simulink model "test_CHCmdApi1"  (R2023a)
settings: Solver=ode4  StartTime=0.0  StopTime=10.0  FixedStep=0.002  RelTol=1e-3
libraries: AFC5Toolbox x6
settings Model: Creator=zhangr365  LastModifiedBy=zqinghua
settings OptimizationCC: DefaultParameterBehavior=Inlined  EnhancedBackFolding=on  PassReuseOutputArgsAs=Individual arguments  ZeroExternalMemoryAtStartup=off  ZeroInternalMemoryAtStartup=off  OptimizeBlockOrder=speed  DifferentSizesBufferReuse=on  OptimizationCustomize=off  EfficientTunableParamExpr=on
settings DebuggingCC: ParameterTunabilityLossMsg=error
settings HardwareCC: ProdBitPerInt=16  ProdBitPerPointer=16  ProdBitPerSizeT=16  ProdBitPerPtrDiffT=16  ProdLargestAtomicFloat=None  ProdWordSize=16  ProdHWDeviceType=STMicroelectronics->ST10/Super10
settings SFSimCC: MATLABDynamicMemAlloc=off
settings RTWCC: Description=Embedded Coder  SystemTargetFile=AFCHawk.tlc  GenCodeOnly=on  TemplateMakefile=ert_default_tmf
settings CodeAppCC: ForceParamTrailComments=on  IgnoreCustomStorageClasses=off  OperatorAnnotations=on  SimulinkDataObjDesc=on  SFDataObjDesc=on  InsertBlockDesc=on
settings STFCustomTargetCC: MultiwordLength=256  ModelReferenceCompliant=off  ConcurrentExecutionCompliant=off  CombineOutputUpdateFcns=on  ERTCustomFileBanners=on  SupportContinuousTime=off  SupportNonInlinedSFcns=off  RemoveResetFunc=on  MATLABClassNameForMDSCustomization=Simulink.SoftwareTarget.ERTCustomization  GRTInterface=off  UseToolchainInfoCompliant=off  SystemTargetFile=AFCHawk.tlc
settings ERTTargetCC: TargetLangStandard=C99 (ISO)  ModelReferenceCompliant=off  ParMdlRefBuildCompliant=off  CompOptLevelCompliant=off  ConcurrentExecutionCompliant=off  ModelStepFunctionPrototypeControlCompliant=off  CPPClassGenCompliant=off  UseToolchainInfoCompliant=off  InlinedParameterPlacement=NonHierarchical  ERTCustomFileTemplate=example_file_process.tlc

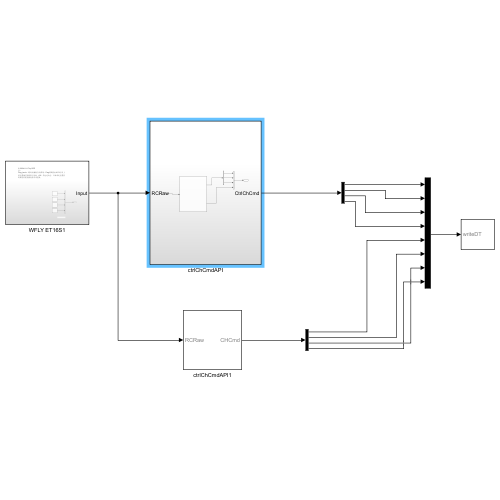
[thumbnail: Simulink's stored preview of the top-level diagram]
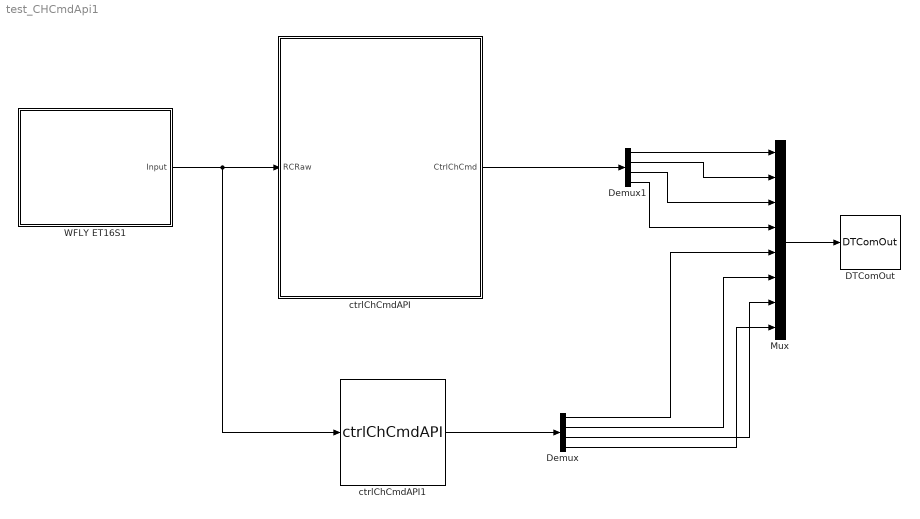
== system test_CHCmdApi1 ==
  DTComOut : AFC5Toolbox/DeviceModule/DTComOut  Priority=8  g_frameType=1  g_outFreq=1  g_comPort=0  g_instName=0  g_id=0
      settings: SourceProductName=AFC5Toolbox
  Demux : Demux
  Demux1 : Demux
  Mux : Mux  Inputs=8
  WFLY ET16S1 : Subsystem  Priority=0
  ctrlChCmdAPI : Subsystem
  ctrlChCmdAPI1 : AFC5Toolbox/APPModule/ctrlChCmdAPI  Priority=3
      settings: SourceProductName=AFC5Toolbox
  wires:
  WFLY ET16S1/1(Input) -> ctrlChCmdAPI1/1, ctrlChCmdAPI/1(RCRaw)
  ctrlChCmdAPI1/1 -> Demux/1
  ctrlChCmdAPI/1(CtrlChCmd) -> Demux1/1
  Demux1/1 -> Mux/1
  Demux1/2 -> Mux/2
  Demux1/3 -> Mux/3
  Demux1/4 -> Mux/4
  Demux/1 -> Mux/5
  Demux/2 -> Mux/6
  Demux/3 -> Mux/7
  Demux/4 -> Mux/8
  Mux/1 -> DTComOut/1

== system test_CHCmdApi1/WFLY ET16S1 ==
  note: cmd4 = [352,1695]
  note: % 2024-01-17 by REZ
      | 注：
      | Flag_land = 1的时候触发自动降落，Flag的跳变由X和Y方向上的位置偏差距离原点坐标（0,0）的远近决定，具体参见位置控制器里的航迹规划指令设置处
  Mux2 : Mux
  SBusCmd{,1..3} (4 alike) : AFC5Toolbox/DeviceModule/SBusCmd  Priority=0  g_SBusChanel=1  g_sampleTime=0.002
      settings: SourceProductName=AFC5Toolbox
  Input : Outport
  wires:
  Mux2/1 -> Input/1
  SBusCmd3/1 -> Mux2/4
  SBusCmd/1 -> Mux2/1
  SBusCmd1/1 -> Mux2/2
  SBusCmd2/1 -> Mux2/3

== system test_CHCmdApi1/ctrlChCmdAPI ==
  RCRaw : Inport
  Demux : Demux  Outputs=3
  Mux : Mux
  get_rccmd_simulink_value : Subsystem
  CtrlChCmd : Outport
  wires:
  RCRaw/1 -> get_rccmd_simulink_value/1(RCRaw)
  get_rccmd_simulink_value/1(RCServCmd) -> Demux/1
  Demux/1 -> Mux/1
  Demux/2 -> Mux/2
  Demux/3 -> Mux/3
  get_rccmd_simulink_value/2(climb_rate) -> Mux/4
  Mux/1 -> CtrlChCmd/1

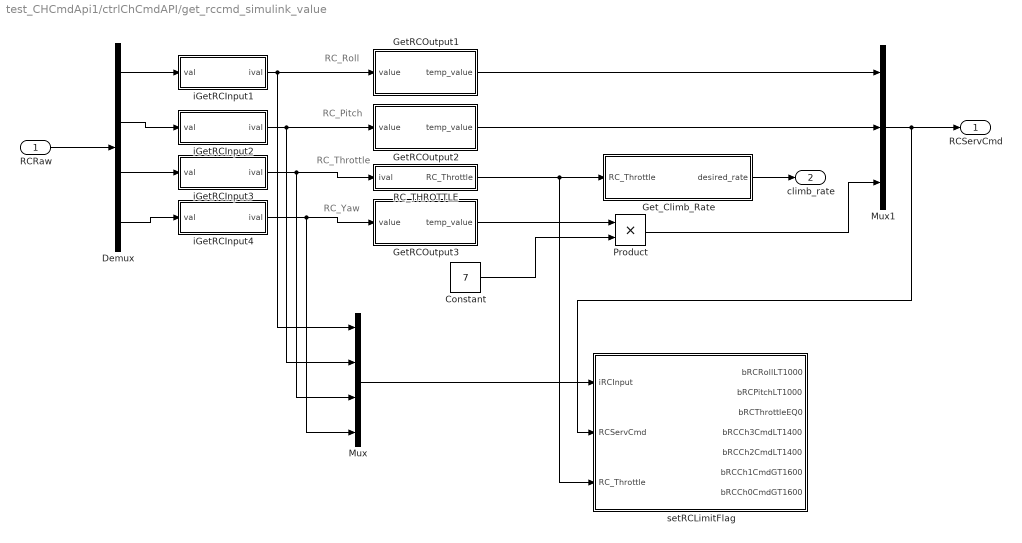
== system test_CHCmdApi1/ctrlChCmdAPI/get_rccmd_simulink_value ==
  note: RC_Roll
  note: RC_Pitch
  note: RC_Yaw
  note: RC_Throttle
  RCRaw : Inport
  Constant : Constant  Value=7
  Demux : Demux
  GetRCOutput1 : Subsystem
  GetRCOutput2 : Subsystem
  GetRCOutput3 : Subsystem
  Get_Climb_Rate : Subsystem
  Mux : Mux
  Mux1 : Mux  Inputs=3
  Product : Product
  RC_THROTTLE : Subsystem
  iGetRCInput1 : Subsystem
  iGetRCInput2 : Subsystem
  iGetRCInput3 : Subsystem
  iGetRCInput4 : Subsystem
  setRCLimitFlag : Subsystem
  RCServCmd : Outport
  climb_rate : Outport  Port=2
  wires:
  Demux/3 -> iGetRCInput3/1(val)
  Demux/4 -> iGetRCInput4/1(val)
  RCRaw/1 -> Demux/1
  Demux/1 -> iGetRCInput1/1(val)
  Mux/1 -> setRCLimitFlag/1(iRCInput)
  GetRCOutput3/1(temp_value) -> Product/1
  Demux/2 -> iGetRCInput2/1(val)
  iGetRCInput4/1(ival) -> Mux/4, GetRCOutput3/1(value)
  iGetRCInput2/1(ival) -> Mux/2, GetRCOutput2/1(value)
  RC_THROTTLE/1(RC_Throttle) -> Get_Climb_Rate/1(RC_Throttle), setRCLimitFlag/3(RC_Throttle)
  iGetRCInput3/1(ival) -> Mux/3, RC_THROTTLE/1(ival)
  Get_Climb_Rate/1(desired_rate) -> climb_rate/1
  iGetRCInput1/1(ival) -> GetRCOutput1/1(value), Mux/1
  Constant/1 -> Product/2
  Product/1 -> Mux1/3
  GetRCOutput1/1(temp_value) -> Mux1/1
  GetRCOutput2/1(temp_value) -> Mux1/2
  Mux1/1 -> RCServCmd/1, setRCLimitFlag/2(RCServCmd)

== system test_CHCmdApi1/ctrlChCmdAPI/get_rccmd_simulink_value/GetRCOutput1 ==
  value : Inport
  If : If  IfExpression=u1 > 1600  ElseIfExpressions=u1 <1400
  If Action Subsystem : Subsystem  TreatAsAtomicUnit=on
  If Action Subsystem1 : Subsystem  TreatAsAtomicUnit=on
  If Action Subsystem2 : Subsystem  TreatAsAtomicUnit=on
  Merge : Merge  Inputs=3
  temp_value : Outport
  wires:
  value/1 -> If Action Subsystem1/1(value), If Action Subsystem/1(value), If/1
  If/1 -> If Action Subsystem/Action
  If/2 -> If Action Subsystem1/Action
  If/3 -> If Action Subsystem2/Action
  If Action Subsystem1/1(temp_value) -> Merge/2
  If Action Subsystem/1(temp_value) -> Merge/1
  If Action Subsystem2/1(temp_value) -> Merge/3
  Merge/1 -> temp_value/1

== system test_CHCmdApi1/ctrlChCmdAPI/get_rccmd_simulink_value/GetRCOutput2 ==
  value : Inport
  If : If  IfExpression=u1 > 1600  ElseIfExpressions=u1 <1400
  If Action Subsystem : Subsystem  TreatAsAtomicUnit=on
  If Action Subsystem1 : Subsystem  TreatAsAtomicUnit=on
  If Action Subsystem2 : Subsystem  TreatAsAtomicUnit=on
  Merge : Merge  Inputs=3
  temp_value : Outport
  wires:
  value/1 -> If Action Subsystem1/1(value), If Action Subsystem/1(value), If/1
  If/1 -> If Action Subsystem/Action
  If/2 -> If Action Subsystem1/Action
  If/3 -> If Action Subsystem2/Action
  If Action Subsystem1/1(temp_value) -> Merge/2
  If Action Subsystem/1(temp_value) -> Merge/1
  If Action Subsystem2/1(temp_value) -> Merge/3
  Merge/1 -> temp_value/1

== system test_CHCmdApi1/ctrlChCmdAPI/get_rccmd_simulink_value/GetRCOutput3 ==
  value : Inport
  If : If  IfExpression=u1 > 1600  ElseIfExpressions=u1 <1400
  If Action Subsystem : Subsystem  TreatAsAtomicUnit=on
  If Action Subsystem1 : Subsystem  TreatAsAtomicUnit=on
  If Action Subsystem2 : Subsystem  TreatAsAtomicUnit=on
  Merge : Merge  Inputs=3
  temp_value : Outport
  wires:
  value/1 -> If Action Subsystem1/1(value), If Action Subsystem/1(value), If/1
  If/1 -> If Action Subsystem/Action
  If/2 -> If Action Subsystem1/Action
  If/3 -> If Action Subsystem2/Action
  If Action Subsystem1/1(temp_value) -> Merge/2
  If Action Subsystem/1(temp_value) -> Merge/1
  If Action Subsystem2/1(temp_value) -> Merge/3
  Merge/1 -> temp_value/1

== system test_CHCmdApi1/ctrlChCmdAPI/get_rccmd_simulink_value/Get_Climb_Rate ==
  RC_Throttle : Inport
  If : If  IfExpression=u1 < 400  ElseIfExpressions=u1 > 600
  If Action Subsystem1 : Subsystem  TreatAsAtomicUnit=on
  If Action Subsystem2 : Subsystem  TreatAsAtomicUnit=on
  If Action Subsystem3 : Subsystem  TreatAsAtomicUnit=on
  Merge : Merge  Inputs=3
  desired_rate : Outport
  wires:
  If Action Subsystem2/1(desired_rate) -> Merge/1
  Merge/1 -> desired_rate/1
  If Action Subsystem3/1(desired_rate) -> Merge/3
  RC_Throttle/1 -> If Action Subsystem2/1(value), If Action Subsystem1/1(value), If/1
  If/1 -> If Action Subsystem2/Action
  If/2 -> If Action Subsystem1/Action
  If/3 -> If Action Subsystem3/Action
  If Action Subsystem1/1(desired_rate) -> Merge/2

== system test_CHCmdApi1/ctrlChCmdAPI/get_rccmd_simulink_value/RC_THROTTLE ==
  ival : Inport
  If : If  IfExpression=u1 < 1100  ElseIfExpressions=u1 > 1900
  If Action Subsystem1 : Subsystem  TreatAsAtomicUnit=on
  If Action Subsystem2 : Subsystem  TreatAsAtomicUnit=on
  If Action Subsystem3 : Subsystem  TreatAsAtomicUnit=on
  Merge : Merge  Inputs=3
  RC_Throttle : Outport
  wires:
  ival/1 -> If Action Subsystem3/1(ival), If/1
  If/1 -> If Action Subsystem2/Action
  If Action Subsystem2/1(RC_Throttle) -> Merge/1
  If/2 -> If Action Subsystem1/Action
  If Action Subsystem1/1(RC_Throttle) -> Merge/2
  If/3 -> If Action Subsystem3/Action
  If Action Subsystem3/1(RC_Throttle) -> Merge/3
  Merge/1 -> RC_Throttle/1

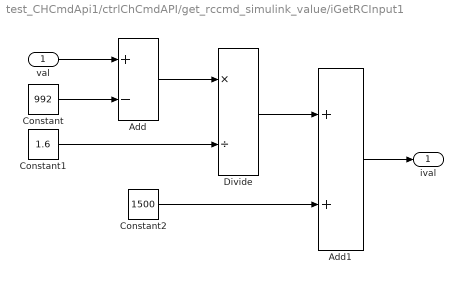
== system test_CHCmdApi1/ctrlChCmdAPI/get_rccmd_simulink_value/iGetRCInput1 ==
  val : Inport
  Add : Sum  Inputs=+-
  Add1 : Sum
  Constant : Constant  Value=992
  Constant1 : Constant  Value=1.6
  Constant2 : Constant  Value=1500
  Divide : Product  Inputs=*/
  ival : Outport
  wires:
  val/1 -> Add/1
  Constant/1 -> Add/2
  Add/1 -> Divide/1
  Constant1/1 -> Divide/2
  Divide/1 -> Add1/1
  Constant2/1 -> Add1/2
  Add1/1 -> ival/1

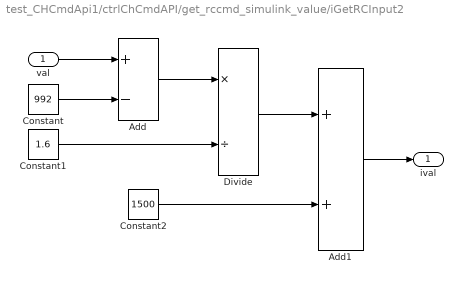
== system test_CHCmdApi1/ctrlChCmdAPI/get_rccmd_simulink_value/iGetRCInput2 ==
  val : Inport
  Add : Sum  Inputs=+-
  Add1 : Sum
  Constant : Constant  Value=992
  Constant1 : Constant  Value=1.6
  Constant2 : Constant  Value=1500
  Divide : Product  Inputs=*/
  ival : Outport
  wires:
  val/1 -> Add/1
  Constant/1 -> Add/2
  Add/1 -> Divide/1
  Constant1/1 -> Divide/2
  Divide/1 -> Add1/1
  Constant2/1 -> Add1/2
  Add1/1 -> ival/1

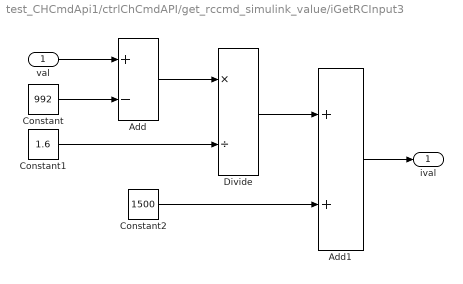
== system test_CHCmdApi1/ctrlChCmdAPI/get_rccmd_simulink_value/iGetRCInput3 ==
  val : Inport
  Add : Sum  Inputs=+-
  Add1 : Sum
  Constant : Constant  Value=992
  Constant1 : Constant  Value=1.6
  Constant2 : Constant  Value=1500
  Divide : Product  Inputs=*/
  ival : Outport
  wires:
  val/1 -> Add/1
  Constant/1 -> Add/2
  Add/1 -> Divide/1
  Constant1/1 -> Divide/2
  Divide/1 -> Add1/1
  Constant2/1 -> Add1/2
  Add1/1 -> ival/1

== system test_CHCmdApi1/ctrlChCmdAPI/get_rccmd_simulink_value/iGetRCInput4 ==
  val : Inport
  Add : Sum  Inputs=+-
  Add1 : Sum
  Constant : Constant  Value=992
  Constant1 : Constant  Value=1.6
  Constant2 : Constant  Value=1500
  Divide : Product  Inputs=*/
  ival : Outport
  wires:
  val/1 -> Add/1
  Constant/1 -> Add/2
  Add/1 -> Divide/1
  Constant1/1 -> Divide/2
  Divide/1 -> Add1/1
  Constant2/1 -> Add1/2
  Add1/1 -> ival/1

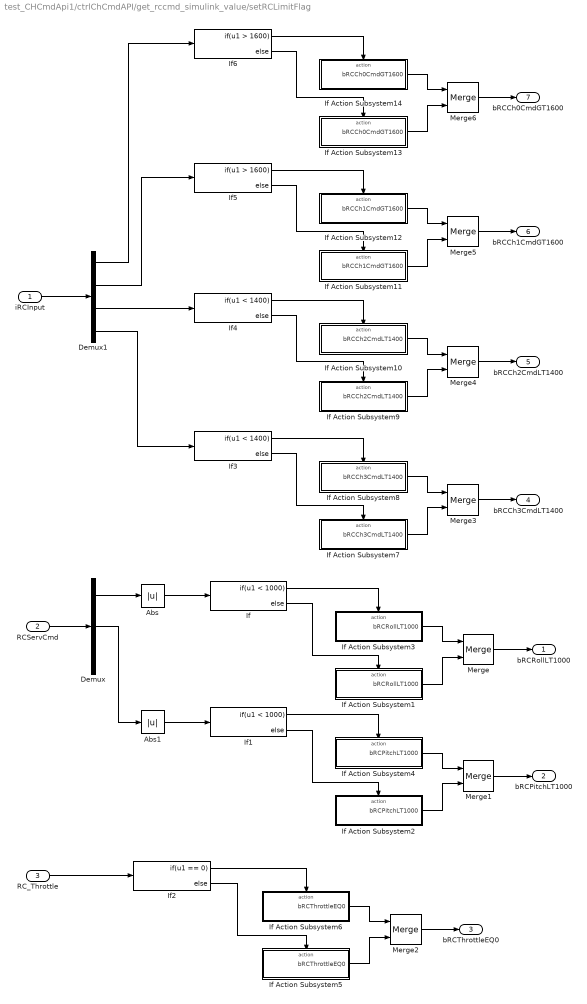
== system test_CHCmdApi1/ctrlChCmdAPI/get_rccmd_simulink_value/setRCLimitFlag ==
  iRCInput : Inport
  RCServCmd : Inport  Port=2
  RC_Throttle : Inport  Port=3
  Abs : Abs  SaturateOnIntegerOverflow=off
  Abs1 : Abs  SaturateOnIntegerOverflow=off
  Demux : Demux  Outputs=3
  Demux1 : Demux
  If : If  IfExpression=u1 < 1000
  If Action Subsystem1 : Subsystem  TreatAsAtomicUnit=on
  If Action Subsystem10 : Subsystem  TreatAsAtomicUnit=on
  If Action Subsystem11 : Subsystem  TreatAsAtomicUnit=on
  If Action Subsystem12 : Subsystem  TreatAsAtomicUnit=on
  If Action Subsystem13 : Subsystem  TreatAsAtomicUnit=on
  If Action Subsystem14 : Subsystem  TreatAsAtomicUnit=on
  If Action Subsystem2 : Subsystem  TreatAsAtomicUnit=on
  If Action Subsystem3 : Subsystem  TreatAsAtomicUnit=on
  If Action Subsystem4 : Subsystem  TreatAsAtomicUnit=on
  If Action Subsystem5 : Subsystem  TreatAsAtomicUnit=on
  If Action Subsystem6 : Subsystem  TreatAsAtomicUnit=on
  If Action Subsystem7 : Subsystem  TreatAsAtomicUnit=on
  If Action Subsystem8 : Subsystem  TreatAsAtomicUnit=on
  If Action Subsystem9 : Subsystem  TreatAsAtomicUnit=on
  If1 : If  IfExpression=u1 < 1000
  If2 : If  IfExpression=u1 == 0
  If3 : If  IfExpression=u1 < 1400
  If4 : If  IfExpression=u1 < 1400
  If5 : If  IfExpression=u1 > 1600
  If6 : If  IfExpression=u1 > 1600
  Merge{,1..6} (7 alike) : Merge
  bRCRollLT1000 : Outport
  bRCPitchLT1000 : Outport  Port=2
  bRCThrottleEQ0 : Outport  Port=3
  bRCCh3CmdLT1400 : Outport  Port=4
  bRCCh2CmdLT1400 : Outport  Port=5
  bRCCh1CmdGT1600 : Outport  Port=6
  bRCCh0CmdGT1600 : Outport  Port=7
  wires:
  RCServCmd/1 -> Demux/1
  Demux/1 -> Abs/1
  Abs/1 -> If/1
  If/1 -> If Action Subsystem3/Action
  If/2 -> If Action Subsystem1/Action
  If Action Subsystem3/1(bRCRollLT1000) -> Merge/1
  If Action Subsystem1/1(bRCRollLT1000) -> Merge/2
  Merge/1 -> bRCRollLT1000/1
  If Action Subsystem2/1(bRCPitchLT1000) -> Merge1/2
  If1/1 -> If Action Subsystem4/Action
  Merge1/1 -> bRCPitchLT1000/1
  If Action Subsystem4/1(bRCPitchLT1000) -> Merge1/1
  If1/2 -> If Action Subsystem2/Action
  Abs1/1 -> If1/1
  Demux/2 -> Abs1/1
  RC_Throttle/1 -> If2/1
  If2/2 -> If Action Subsystem5/Action
  If2/1 -> If Action Subsystem6/Action
  If Action Subsystem5/1(bRCThrottleEQ0) -> Merge2/2
  Merge2/1 -> bRCThrottleEQ0/1
  If Action Subsystem6/1(bRCThrottleEQ0) -> Merge2/1
  iRCInput/1 -> Demux1/1
  If Action Subsystem7/1(bRCCh3CmdLT1400) -> Merge3/2
  Merge3/1 -> bRCCh3CmdLT1400/1
  If Action Subsystem8/1(bRCCh3CmdLT1400) -> Merge3/1
  Demux1/4 -> If3/1
  If Action Subsystem9/1(bRCCh2CmdLT1400) -> Merge4/2
  Merge4/1 -> bRCCh2CmdLT1400/1
  If Action Subsystem10/1(bRCCh2CmdLT1400) -> Merge4/1
  Demux1/3 -> If4/1
  If Action Subsystem11/1(bRCCh1CmdGT1600) -> Merge5/2
  Merge5/1 -> bRCCh1CmdGT1600/1
  If Action Subsystem12/1(bRCCh1CmdGT1600) -> Merge5/1
  Demux1/2 -> If5/1
  If Action Subsystem13/1(bRCCh0CmdGT1600) -> Merge6/2
  Merge6/1 -> bRCCh0CmdGT1600/1
  If Action Subsystem14/1(bRCCh0CmdGT1600) -> Merge6/1
  Demux1/1 -> If6/1
  If6/1 -> If Action Subsystem14/Action
  If6/2 -> If Action Subsystem13/Action
  If5/1 -> If Action Subsystem12/Action
  If5/2 -> If Action Subsystem11/Action
  If4/1 -> If Action Subsystem10/Action
  If4/2 -> If Action Subsystem9/Action
  If3/1 -> If Action Subsystem8/Action
  If3/2 -> If Action Subsystem7/Action

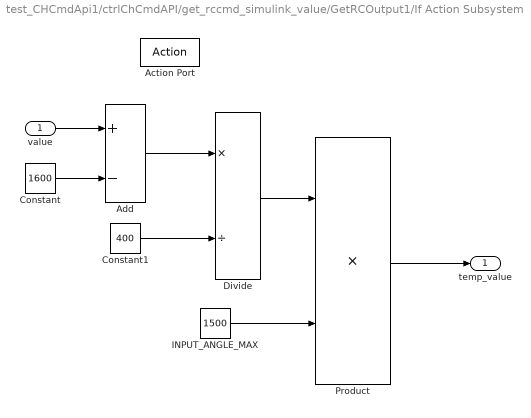
== system test_CHCmdApi1/ctrlChCmdAPI/get_rccmd_simulink_value/GetRCOutput1/If Action Subsystem ==
  value : Inport
  Action Port : ActionPort  ActionPortLabel=if(u1 > 1600)
  Add : Sum  Inputs=+-
  Constant : Constant  Value=1600
  Constant1 : Constant  Value=400
  Divide : Product  Inputs=*/
  INPUT_ANGLE_MAX : Constant  Value=1500
  Product : Product
  temp_value : Outport
  wires:
  value/1 -> Add/1
  Constant/1 -> Add/2
  Add/1 -> Divide/1
  Constant1/1 -> Divide/2
  Divide/1 -> Product/1
  INPUT_ANGLE_MAX/1 -> Product/2
  Product/1 -> temp_value/1

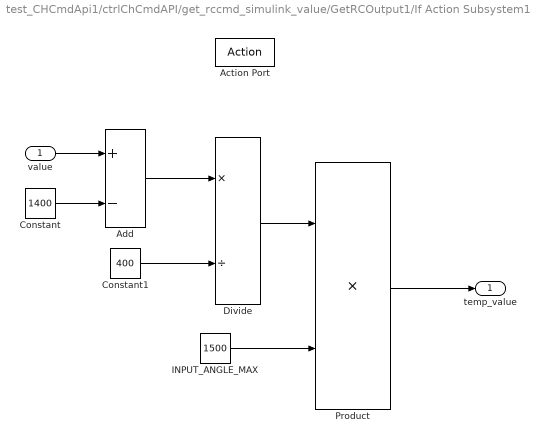
== system test_CHCmdApi1/ctrlChCmdAPI/get_rccmd_simulink_value/GetRCOutput1/If Action Subsystem1 ==
  value : Inport
  Action Port : ActionPort  ActionPortLabel=elseif(u1 <1400)
  Add : Sum  Inputs=+-
  Constant : Constant  Value=1400
  Constant1 : Constant  Value=400
  Divide : Product  Inputs=*/
  INPUT_ANGLE_MAX : Constant  Value=1500
  Product : Product
  temp_value : Outport
  wires:
  INPUT_ANGLE_MAX/1 -> Product/2
  Constant1/1 -> Divide/2
  Add/1 -> Divide/1
  value/1 -> Add/1
  Product/1 -> temp_value/1
  Constant/1 -> Add/2
  Divide/1 -> Product/1

== system test_CHCmdApi1/ctrlChCmdAPI/get_rccmd_simulink_value/GetRCOutput1/If Action Subsystem2 ==
  Action Port : ActionPort  ActionPortLabel=else
  Constant : Constant  Value=0
  temp_value : Outport
  wires:
  Constant/1 -> temp_value/1

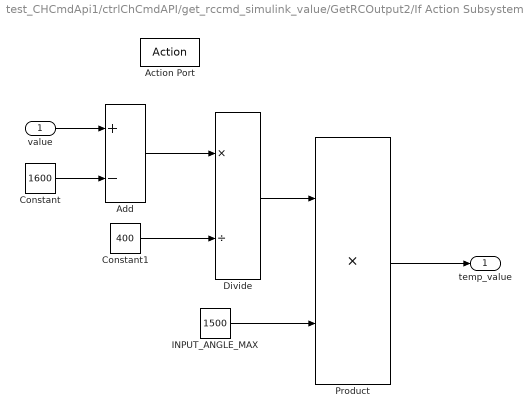
== system test_CHCmdApi1/ctrlChCmdAPI/get_rccmd_simulink_value/GetRCOutput2/If Action Subsystem ==
  value : Inport
  Action Port : ActionPort  ActionPortLabel=if(u1 > 1600)
  Add : Sum  Inputs=+-
  Constant : Constant  Value=1600
  Constant1 : Constant  Value=400
  Divide : Product  Inputs=*/
  INPUT_ANGLE_MAX : Constant  Value=1500
  Product : Product
  temp_value : Outport
  wires:
  value/1 -> Add/1
  Constant/1 -> Add/2
  Add/1 -> Divide/1
  Constant1/1 -> Divide/2
  Divide/1 -> Product/1
  INPUT_ANGLE_MAX/1 -> Product/2
  Product/1 -> temp_value/1

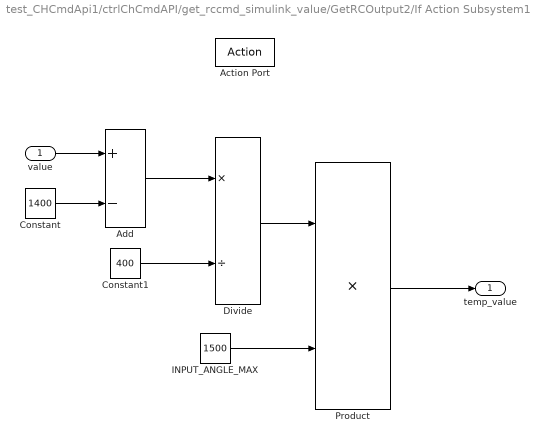
== system test_CHCmdApi1/ctrlChCmdAPI/get_rccmd_simulink_value/GetRCOutput2/If Action Subsystem1 ==
  value : Inport
  Action Port : ActionPort  ActionPortLabel=elseif(u1 <1400)
  Add : Sum  Inputs=+-
  Constant : Constant  Value=1400
  Constant1 : Constant  Value=400
  Divide : Product  Inputs=*/
  INPUT_ANGLE_MAX : Constant  Value=1500
  Product : Product
  temp_value : Outport
  wires:
  INPUT_ANGLE_MAX/1 -> Product/2
  Constant1/1 -> Divide/2
  Add/1 -> Divide/1
  value/1 -> Add/1
  Product/1 -> temp_value/1
  Constant/1 -> Add/2
  Divide/1 -> Product/1

== system test_CHCmdApi1/ctrlChCmdAPI/get_rccmd_simulink_value/GetRCOutput2/If Action Subsystem2 ==
  Action Port : ActionPort  ActionPortLabel=else
  Constant : Constant  Value=0
  temp_value : Outport
  wires:
  Constant/1 -> temp_value/1

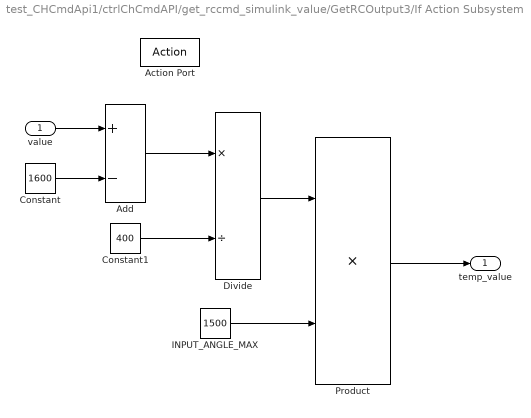
== system test_CHCmdApi1/ctrlChCmdAPI/get_rccmd_simulink_value/GetRCOutput3/If Action Subsystem ==
  value : Inport
  Action Port : ActionPort  ActionPortLabel=if(u1 > 1600)
  Add : Sum  Inputs=+-
  Constant : Constant  Value=1600
  Constant1 : Constant  Value=400
  Divide : Product  Inputs=*/
  INPUT_ANGLE_MAX : Constant  Value=1500
  Product : Product
  temp_value : Outport
  wires:
  value/1 -> Add/1
  Constant/1 -> Add/2
  Add/1 -> Divide/1
  Constant1/1 -> Divide/2
  Divide/1 -> Product/1
  INPUT_ANGLE_MAX/1 -> Product/2
  Product/1 -> temp_value/1

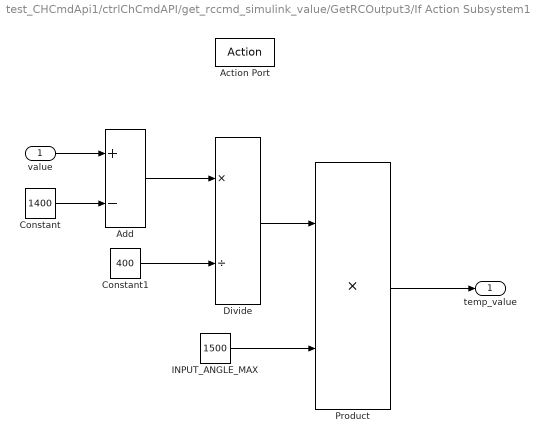
== system test_CHCmdApi1/ctrlChCmdAPI/get_rccmd_simulink_value/GetRCOutput3/If Action Subsystem1 ==
  value : Inport
  Action Port : ActionPort  ActionPortLabel=elseif(u1 <1400)
  Add : Sum  Inputs=+-
  Constant : Constant  Value=1400
  Constant1 : Constant  Value=400
  Divide : Product  Inputs=*/
  INPUT_ANGLE_MAX : Constant  Value=1500
  Product : Product
  temp_value : Outport
  wires:
  INPUT_ANGLE_MAX/1 -> Product/2
  Constant1/1 -> Divide/2
  Add/1 -> Divide/1
  value/1 -> Add/1
  Product/1 -> temp_value/1
  Constant/1 -> Add/2
  Divide/1 -> Product/1

== system test_CHCmdApi1/ctrlChCmdAPI/get_rccmd_simulink_value/GetRCOutput3/If Action Subsystem2 ==
  Action Port : ActionPort  ActionPortLabel=else
  Constant : Constant  Value=0
  temp_value : Outport
  wires:
  Constant/1 -> temp_value/1

== system test_CHCmdApi1/ctrlChCmdAPI/get_rccmd_simulink_value/Get_Climb_Rate/If Action Subsystem1 ==
  value : Inport
  Action Port : ActionPort  ActionPortLabel=elseif(u1 > 600)
  Add : Sum  Inputs=+-
  Constant : Constant  Value=600
  Constant1 : Constant  Value=250
  Constant2 : Constant  Value=400
  Divide : Product  Inputs=**/
  desired_rate : Outport
  wires:
  Constant/1 -> Add/2
  Constant1/1 -> Divide/2
  Add/1 -> Divide/1
  Constant2/1 -> Divide/3
  Divide/1 -> desired_rate/1
  value/1 -> Add/1

== system test_CHCmdApi1/ctrlChCmdAPI/get_rccmd_simulink_value/Get_Climb_Rate/If Action Subsystem2 ==
  value : Inport
  Action Port : ActionPort  ActionPortLabel=if(u1 < 400)
  Add : Sum  Inputs=+-
  Constant : Constant  Value=400
  Constant1 : Constant  Value=250
  Constant2 : Constant  Value=400
  Divide : Product  Inputs=**/
  desired_rate : Outport
  wires:
  value/1 -> Add/1
  Constant/1 -> Add/2
  Add/1 -> Divide/1
  Divide/1 -> desired_rate/1
  Constant1/1 -> Divide/2
  Constant2/1 -> Divide/3

== system test_CHCmdApi1/ctrlChCmdAPI/get_rccmd_simulink_value/Get_Climb_Rate/If Action Subsystem3 ==
  Action Port : ActionPort  ActionPortLabel=else
  Constant : Constant  Value=0
  desired_rate : Outport
  wires:
  Constant/1 -> desired_rate/1

== system test_CHCmdApi1/ctrlChCmdAPI/get_rccmd_simulink_value/RC_THROTTLE/If Action Subsystem1 ==
  Action Port : ActionPort  ActionPortLabel=elseif(u1 > 1900)
  Constant : Constant  Value=1000
  RC_Throttle : Outport
  wires:
  Constant/1 -> RC_Throttle/1

== system test_CHCmdApi1/ctrlChCmdAPI/get_rccmd_simulink_value/RC_THROTTLE/If Action Subsystem2 ==
  Action Port : ActionPort  ActionPortLabel=if(u1 < 1100)
  Constant : Constant  Value=0
  RC_Throttle : Outport
  wires:
  Constant/1 -> RC_Throttle/1

== system test_CHCmdApi1/ctrlChCmdAPI/get_rccmd_simulink_value/RC_THROTTLE/If Action Subsystem3 ==
  ival : Inport
  Action Port : ActionPort  ActionPortLabel=else
  Add : Sum  Inputs=+-
  Constant : Constant  Value=1100
  Constant1 : Constant  Value=1.25
  Product : Product
  RC_Throttle : Outport
  wires:
  ival/1 -> Add/1
  Constant/1 -> Add/2
  Add/1 -> Product/1
  Constant1/1 -> Product/2
  Product/1 -> RC_Throttle/1

== system test_CHCmdApi1/ctrlChCmdAPI/get_rccmd_simulink_value/setRCLimitFlag/If Action Subsystem1 ==
  Action Port : ActionPort  ActionPortLabel=else
  Constant : Constant  Value=0
  bRCRollLT1000 : Outport
  wires:
  Constant/1 -> bRCRollLT1000/1

== system test_CHCmdApi1/ctrlChCmdAPI/get_rccmd_simulink_value/setRCLimitFlag/If Action Subsystem10 ==
  Action Port : ActionPort  ActionPortLabel=if(u1 < 1400)
  Constant : Constant
  bRCCh2CmdLT1400 : Outport
  wires:
  Constant/1 -> bRCCh2CmdLT1400/1

== system test_CHCmdApi1/ctrlChCmdAPI/get_rccmd_simulink_value/setRCLimitFlag/If Action Subsystem11 ==
  Action Port : ActionPort  ActionPortLabel=else
  Constant : Constant  Value=0
  bRCCh1CmdGT1600 : Outport
  wires:
  Constant/1 -> bRCCh1CmdGT1600/1

== system test_CHCmdApi1/ctrlChCmdAPI/get_rccmd_simulink_value/setRCLimitFlag/If Action Subsystem12 ==
  Action Port : ActionPort  ActionPortLabel=if(u1 > 1600)
  Constant : Constant
  bRCCh1CmdGT1600 : Outport
  wires:
  Constant/1 -> bRCCh1CmdGT1600/1

== system test_CHCmdApi1/ctrlChCmdAPI/get_rccmd_simulink_value/setRCLimitFlag/If Action Subsystem13 ==
  Action Port : ActionPort  ActionPortLabel=else
  Constant : Constant  Value=0
  bRCCh0CmdGT1600 : Outport
  wires:
  Constant/1 -> bRCCh0CmdGT1600/1

== system test_CHCmdApi1/ctrlChCmdAPI/get_rccmd_simulink_value/setRCLimitFlag/If Action Subsystem14 ==
  Action Port : ActionPort  ActionPortLabel=if(u1 > 1600)
  Constant : Constant
  bRCCh0CmdGT1600 : Outport
  wires:
  Constant/1 -> bRCCh0CmdGT1600/1

== system test_CHCmdApi1/ctrlChCmdAPI/get_rccmd_simulink_value/setRCLimitFlag/If Action Subsystem2 ==
  Action Port : ActionPort  ActionPortLabel=else
  Constant : Constant  Value=0
  bRCPitchLT1000 : Outport
  wires:
  Constant/1 -> bRCPitchLT1000/1

== system test_CHCmdApi1/ctrlChCmdAPI/get_rccmd_simulink_value/setRCLimitFlag/If Action Subsystem3 ==
  Action Port : ActionPort  ActionPortLabel=if(u1 < 1000)
  Constant : Constant
  bRCRollLT1000 : Outport
  wires:
  Constant/1 -> bRCRollLT1000/1

== system test_CHCmdApi1/ctrlChCmdAPI/get_rccmd_simulink_value/setRCLimitFlag/If Action Subsystem4 ==
  Action Port : ActionPort  ActionPortLabel=if(u1 < 1000)
  Constant : Constant
  bRCPitchLT1000 : Outport
  wires:
  Constant/1 -> bRCPitchLT1000/1

== system test_CHCmdApi1/ctrlChCmdAPI/get_rccmd_simulink_value/setRCLimitFlag/If Action Subsystem5 ==
  Action Port : ActionPort  ActionPortLabel=else
  Constant : Constant  Value=0
  bRCThrottleEQ0 : Outport
  wires:
  Constant/1 -> bRCThrottleEQ0/1

== system test_CHCmdApi1/ctrlChCmdAPI/get_rccmd_simulink_value/setRCLimitFlag/If Action Subsystem6 ==
  Action Port : ActionPort  ActionPortLabel=if(u1 == 0)
  Constant : Constant
  bRCThrottleEQ0 : Outport
  wires:
  Constant/1 -> bRCThrottleEQ0/1

== system test_CHCmdApi1/ctrlChCmdAPI/get_rccmd_simulink_value/setRCLimitFlag/If Action Subsystem7 ==
  Action Port : ActionPort  ActionPortLabel=else
  Constant : Constant  Value=0
  bRCCh3CmdLT1400 : Outport
  wires:
  Constant/1 -> bRCCh3CmdLT1400/1

== system test_CHCmdApi1/ctrlChCmdAPI/get_rccmd_simulink_value/setRCLimitFlag/If Action Subsystem8 ==
  Action Port : ActionPort  ActionPortLabel=if(u1 < 1400)
  Constant : Constant
  bRCCh3CmdLT1400 : Outport
  wires:
  Constant/1 -> bRCCh3CmdLT1400/1

== system test_CHCmdApi1/ctrlChCmdAPI/get_rccmd_simulink_value/setRCLimitFlag/If Action Subsystem9 ==
  Action Port : ActionPort  ActionPortLabel=else
  Constant : Constant  Value=0
  bRCCh2CmdLT1400 : Outport
  wires:
  Constant/1 -> bRCCh2CmdLT1400/1
